simulink model "NEPTUN_ZH_Z3"  (R2026a)
settings: Solver=VariableStepAuto  StopTime=2  MaxStep=0.1/25
libraries: simulink_extras x1
settings Model: Creator=Szalay  LastModifiedBy=Szalay

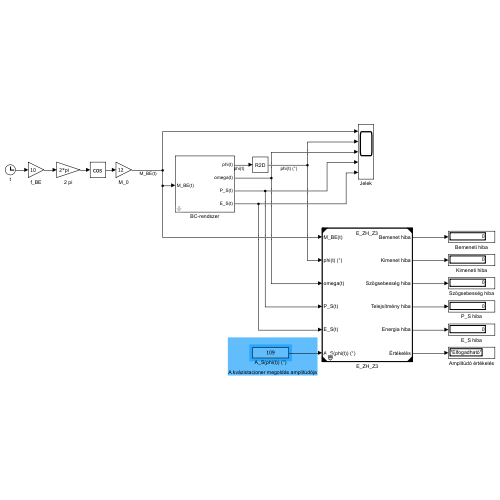
[thumbnail: Simulink's stored preview of the top-level diagram]
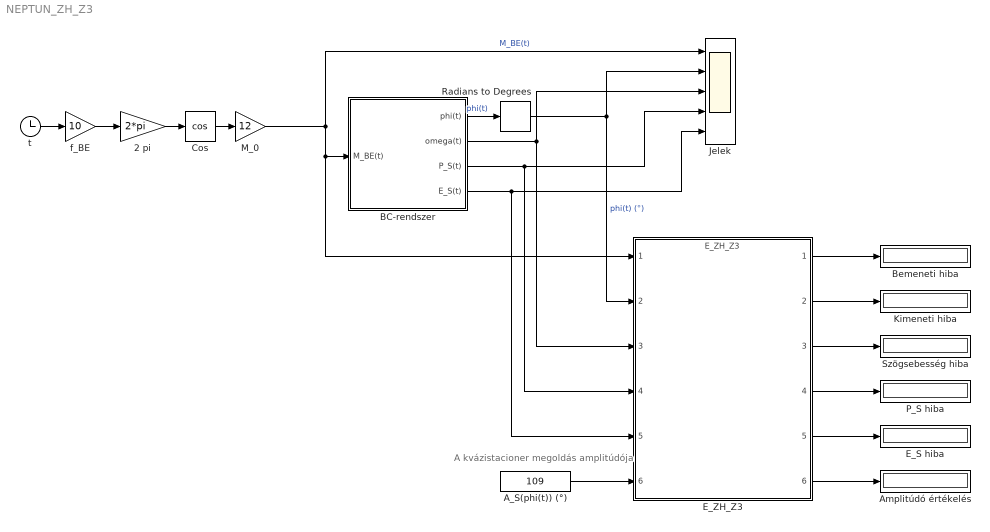
== system NEPTUN_ZH_Z3 ==
  note: A kvázistacioner megoldás amplitúdója
  2 pi : Gain  Gain=2*pi
  A_S(phi(t)) (°) : Constant  Value=109
  Amplitúdó értékelés : Display
  BC-rendszer : Subsystem  mask(BC-rendszer){C=0.5, B=0.1, phi_0=deg2rad(45)}
      mask prompts: C "Csavarási rugómerevség"; B "Forgási súrlódási együttható"; phi_0 "Kezdeti szöghelyzet"
      mask help: A csigarugó ellenében forgó súrlódó tengely.
      mask DialogControl ParameterGroupVar Prompt: Modellparaméterek
      mask DialogControl Container3 Prompt: Kezdeti érték
  Bemeneti hiba : Display
  Cos : Trigonometry  Operator=cos
  E_S hiba : Display
  E_ZH_Z3 : ModelReference  ModelNameDialog=E_ZH_Z3.slxp  ModelReferenceVersion=3.4  CopyOfModelProtected=on
  Jelek : Scope  NumInputPorts=5
      settings: ActiveDisplayYMinimum=-14.999941283406589  ActiveDisplayYMaximum=14.999993475934065
  Kimeneti hiba : Display
  M_0 : Gain  Gain=12
  P_S hiba : Display
  Radians to Degrees : simulink_extras/Transformations/Radians to Degrees
  Szögsebesség hiba : Display
  f_BE : Gain  Gain=10
  t : Clock
  wires:
  E_ZH_Z3/1 -> Bemeneti hiba/1
  E_ZH_Z3/2 -> Kimeneti hiba/1
  A_S(phi(t)) (°)/1 -> E_ZH_Z3/6
  E_ZH_Z3/3 -> Szögsebesség hiba/1
  E_ZH_Z3/4 -> P_S hiba/1
  E_ZH_Z3/5 -> E_S hiba/1
  E_ZH_Z3/6 -> Amplitúdó értékelés/1
  BC-rendszer/1(phi(t)) -> Radians to Degrees/1  "phi(t)"
  Radians to Degrees/1 -> E_ZH_Z3/2, Jelek/2  "phi(t) (°)"
  M_0/1 -> E_ZH_Z3/1, BC-rendszer/1(M_BE(t)), Jelek/1  "M_BE(t)"
  Cos/1 -> M_0/1
  2 pi/1 -> Cos/1
  f_BE/1 -> 2 pi/1
  t/1 -> f_BE/1
  BC-rendszer/2(omega(t)) -> E_ZH_Z3/3, Jelek/3
  BC-rendszer/3(P_S(t)) -> E_ZH_Z3/4, Jelek/4
  BC-rendszer/4(E_S(t)) -> E_ZH_Z3/5, Jelek/5

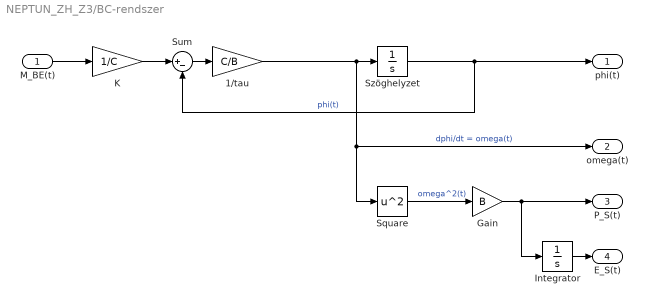
== system NEPTUN_ZH_Z3/BC-rendszer ==
  M_BE(t) : Inport
  1/tau : Gain  Gain=C/B
  Gain : Gain  Gain=B
  Integrator : Integrator
  K : Gain  Gain=1/C
  Square : Math  Operator=square
  Sum : Sum  Inputs=|+-
  Szöghelyzet : Integrator  InitialCondition=phi_0
  phi(t) : Outport
  omega(t) : Outport  Port=2
  P_S(t) : Outport  Port=3
  E_S(t) : Outport  Port=4
  wires:
  K/1 -> Sum/1
  M_BE(t)/1 -> K/1
  Szöghelyzet/1 -> phi(t)/1, Sum/2  "phi(t)"
  Sum/1 -> 1/tau/1
  1/tau/1 -> Square/1, omega(t)/1, Szöghelyzet/1  "dphi/dt = omega(t)"
  Square/1 -> Gain/1  "omega^2(t)"
  Gain/1 -> Integrator/1, P_S(t)/1
  Integrator/1 -> E_S(t)/1
